simulink model "Solar_track_PID"  (R2026b)
settings: Solver=FixedStepAuto  StopTime=60  FixedStep=0.01
InitFcn:
  | Ches_workspace;
values from neighbouring files (symbols this model uses):
  J = J_r + (J_p/N^2)    (= 0.0035)    [Ches_workspace.m]    (also in linsys1.mat = 0.0396; params.m = 0.0396)
  K_a = 0.2    [Ches_workspace.m]    (also in linsys1.mat; params.m)
  K_b = 0.009549    [Ches_workspace.m]    (also in linsys1.mat; params.m)
  K_f = 0.047746    [Ches_workspace.m]    (also in linsys1.mat; params.m)
  K_p = 4    [Ches_workspace.m]    (also in linsys1.mat; params.m)
  K_s = h*(2/1.8)    (= 1.66666666667)    [Ches_workspace.m]    (also in linsys1.mat = 0.277777777778; params.m = 0.277777777778)
  Kd = 15    [Ches_workspace.m]
  Kp = 1    [Ches_workspace.m]
  N = 20    [Ches_workspace.m]    (also in linsys1.mat; params.m)
  R_m = 10    [Ches_workspace.m]    (also in linsys1.mat; params.m)
  Ts = 0.01    [Ches_workspace.m]    (also in linsys1.mat; params.m)
undefined symbols (not defined in the file or in its folder): dspblkCoreblockFVToolHelper, gcbh
settings Model: Creator=milan  LastModifiedBy=moore
settings DataIOCC: ReturnWorkspaceOutputs=off

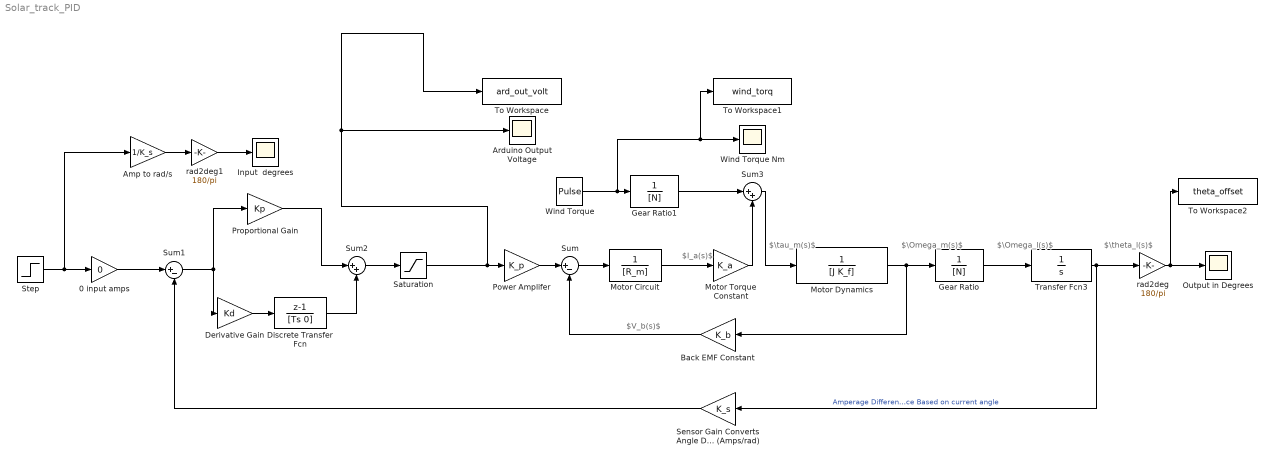
== system Solar_track_PID ==
  note: $V_b(s)$
  note: $I_a(s)$
  note: $\tau_m(s)$
  note: $\Omega_m(s)$
  note: $\Omega_l(s)$
  note: $\theta_l(s)$
  0 input amps : Gain  Gain=0
  Amp to rad/s : Gain  Gain=1/K_s
  Arduino Output Voltage : Scope
      settings: ActiveDisplayYMinimum=-5.625  ActiveDisplayYMaximum=0.62499999999999989  DataLoggingVariableName=ScopeData3
  Back EMF Constant : Gain  Gain=K_b
  Derivative Gain : Gain  Gain=Kd
  Discrete Transfer Fcn : DiscreteTransferFcn  LoadFcn=dspblkCoreblockFVToolHelper(gcbh,'load');  Numerator=[1 -1]  Denominator=[Ts 0]
      settings: CopyFcn=dspblkCoreblockFVToolHelper(gcbh,'copy');  DeleteFcn=dspblkCoreblockFVToolHelper(gcbh,'close');  ModelCloseFcn=dspblkCoreblockFVToolHelper(gcbh,'close');  PreSaveFcn=dspblkCoreblockFVToolHelper(gcbh,'presave');  PostSaveFcn=dspblkCoreblockFVToolHelper(gcbh,'postsave');  CloseFcn=dspblkCoreblockFVToolHelper(gcbh,'close');
  Gear Ratio : TransferFcn  Denominator=[N]
  Gear Ratio1 : TransferFcn  Denominator=[N]
  Input  degrees : Scope
      settings: ActiveDisplayYMinimum=-14.30826241958318  ActiveDisplayYMaximum=86.208767418503754
  Motor Circuit : TransferFcn  Denominator=[R_m]
  Motor Dynamics : TransferFcn  Denominator=[J K_f]
  Motor Torque Constant : Gain  Gain=K_a
  Output in Degrees : Scope
      settings: ActiveDisplayYMinimum=-31.546571750036669  ActiveDisplayYMaximum=283.91914575033007
  Power Amplifer : Gain  Gain=K_p
  Proportional Gain : Gain  Gain=Kp
  Saturation : Saturate  UpperLimit=5  LowerLimit=-5
  Sensor Gain Converts Angle Difference into amp difference (Amps/rad) : Gain  Gain=K_s
  Step : Step  Time=0.01  SampleTime=0.01
  Sum : Sum  Inputs=|+-
  Sum1 : Sum  Inputs=|+-
  Sum2 : Sum  Inputs=|++
  Sum3 : Sum  Inputs=|++
  To Workspace : ToWorkspace  VariableName=ard_out_volt  SaveFormat=Timeseries  SampleTime=-1
  To Workspace1 : ToWorkspace  VariableName=wind_torq  SaveFormat=Timeseries  SampleTime=-1
  To Workspace2 : ToWorkspace  VariableName=theta_offset  SaveFormat=Timeseries  SampleTime=-1
  Transfer Fcn3 : TransferFcn  Denominator=[1 0]
  Wind Torque : DiscretePulseGenerator  PulseType=Time based  Amplitude=25  Period=500
  Wind Torque Nm : Scope
      settings: ActiveDisplayYMinimum=-6.2499999999999982  ActiveDisplayYMaximum=56.25  DataLoggingVariableName=ScopeData2
  rad2deg : Gain  Gain=180/pi
  rad2deg1 : Gain  Gain=180/pi
  wires:
  Motor Circuit/1 -> Motor Torque Constant/1
  Motor Torque Constant/1 -> Sum3/2
  Motor Dynamics/1 -> Gear Ratio/1, Back EMF Constant/1
  Gear Ratio/1 -> Transfer Fcn3/1
  Transfer Fcn3/1 -> Sensor Gain Converts Angle Difference into amp difference (Amps/rad)/1, rad2deg/1  "Amperage Difference Based on current angle"
  Back EMF Constant/1 -> Sum/2
  Sum/1 -> Motor Circuit/1
  Derivative Gain/1 -> Discrete Transfer Fcn/1
  Sensor Gain Converts Angle Difference into amp difference (Amps/rad)/1 -> Sum1/2
  Sum1/1 -> Proportional Gain/1, Derivative Gain/1
  Sum2/1 -> Saturation/1
  Discrete Transfer Fcn/1 -> Sum2/2
  Proportional Gain/1 -> Sum2/1
  rad2deg/1 -> To Workspace2/1, Output in Degrees/1
  Power Amplifer/1 -> Sum/1
  Step/1 -> 0 input amps/1, Amp to rad/s/1
  Amp to rad/s/1 -> rad2deg1/1
  rad2deg1/1 -> Input  degrees/1
  0 input amps/1 -> Sum1/1
  Sum3/1 -> Motor Dynamics/1
  Wind Torque/1 -> To Workspace1/1, Wind Torque Nm/1, Gear Ratio1/1
  Gear Ratio1/1 -> Sum3/1
  Saturation/1 -> To Workspace/1, Arduino Output Voltage/1, Power Amplifer/1
